simulink model "lab5_control"  (R2026a)
settings: Solver=ode4  StopTime=T_FIN  FixedStep=1e-4
PreLoadFcn:
  | run(fullfile(fileparts(get_param(bdroot,'FileName')),'parametros.m'));
InitFcn:
  | run(fullfile(fileparts(get_param(bdroot,'FileName')),'parametros.m'));
values from neighbouring files (symbols this model uses):
  a0 = 622.9    [parametros.m]
  a1 = 46.87    [parametros.m]
  b0 = 168.4    [parametros.m]
  Kd = (Pd_s(2) - a1)/b0    [parametros.m]
  Ki = Pd_s(4)/b0    [parametros.m]
  Kp = (Pd_s(3) - a0)/b0    [parametros.m]
  q0_cd = Kd/T + Kp + Ki*T    [parametros.m]
  q0_dd = sol(1)    [parametros.m]
  q1_cd = -2*Kd/T - Kp    [parametros.m]
  q1_dd = sol(2)    [parametros.m]
  q2_cd = Kd/T    [parametros.m]
  q2_dd = sol(3)    [parametros.m]
  R1 = 5    [parametros.m]
  R2 = -5    [parametros.m]
  s0_cd = 0    [parametros.m]
  s0_dd = sol(4)    [parametros.m]
  T = 0.01    [parametros.m]
  T_R1 = 0.1    [parametros.m]
  T_R2 = 1.6    [parametros.m]
  U_MAX = 100 - U0_POS    (= 57.9)    [parametros.m]
  U_MIN = -(100 - U0_NEG)    (= -44.7)    [parametros.m]
settings Model: Creator=PERSONAL  LastModifiedBy=PERSONAL

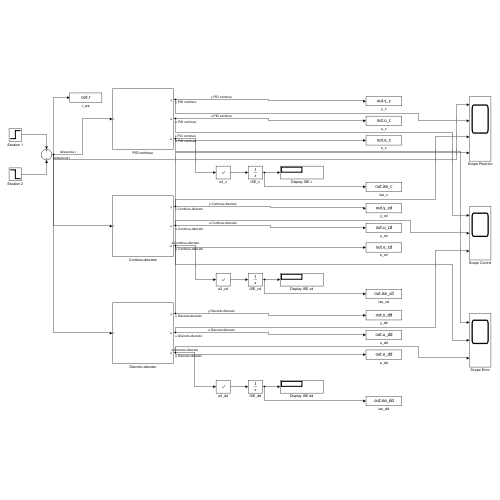
[thumbnail: Simulink's stored preview of the top-level diagram]
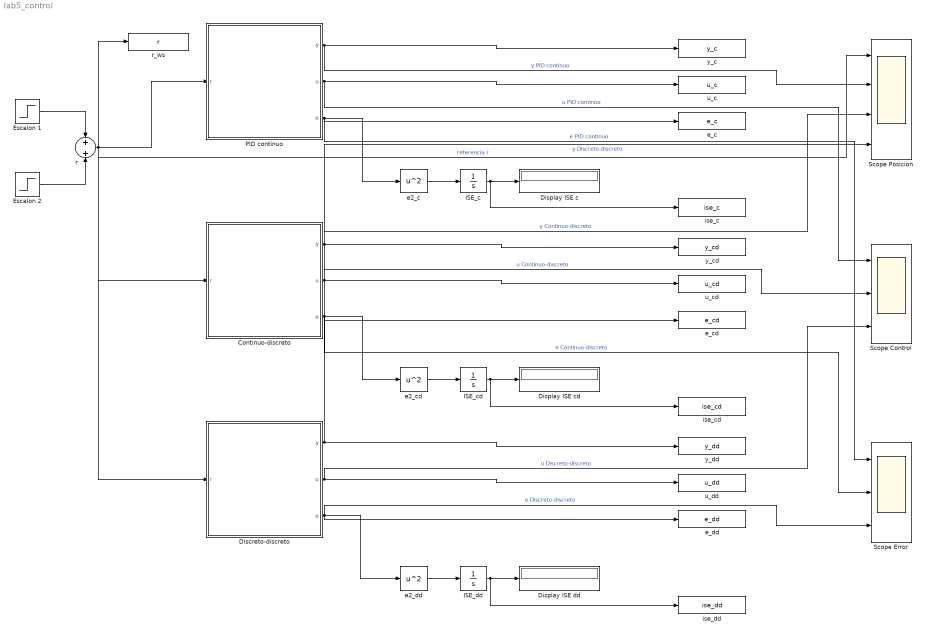
== system lab5_control ==
  Continuo-discreto : Subsystem
  Discreto-discreto : Subsystem
  Display ISE c : Display
  Display ISE cd : Display
  Display ISE dd : Display
  Escalon 1 : Step  Time=T_R1  FinalValue=R1  SampleTime=0
  Escalon 2 : Step  Time=T_R2  FinalValue=R2-R1  SampleTime=0
  ISE_c : Integrator
  ISE_cd : Integrator
  ISE_dd : Integrator
  PID continuo : Subsystem
  Scope Control : Scope  NumInputPorts=3
  Scope Error : Scope  NumInputPorts=3
  Scope Posicion : Scope  NumInputPorts=4
  e2_c : Math  Operator=square
  e2_cd : Math  Operator=square
  e2_dd : Math  Operator=square
  e_c : ToWorkspace  VariableName=e_c  SaveFormat=Timeseries  SampleTime=1e-3
  e_cd : ToWorkspace  VariableName=e_cd  SaveFormat=Timeseries  SampleTime=1e-3
  e_dd : ToWorkspace  VariableName=e_dd  SaveFormat=Timeseries  SampleTime=1e-3
  ise_c : ToWorkspace  VariableName=ise_c  SaveFormat=Timeseries  SampleTime=1e-3
  ise_cd : ToWorkspace  VariableName=ise_cd  SaveFormat=Timeseries  SampleTime=1e-3
  ise_dd : ToWorkspace  VariableName=ise_dd  SaveFormat=Timeseries  SampleTime=1e-3
  r : Sum
  r_ws : ToWorkspace  VariableName=r  SaveFormat=Timeseries  SampleTime=1e-3
  u_c : ToWorkspace  VariableName=u_c  SaveFormat=Timeseries  SampleTime=1e-3
  u_cd : ToWorkspace  VariableName=u_cd  SaveFormat=Timeseries  SampleTime=1e-3
  u_dd : ToWorkspace  VariableName=u_dd  SaveFormat=Timeseries  SampleTime=1e-3
  y_c : ToWorkspace  VariableName=y_c  SaveFormat=Timeseries  SampleTime=1e-3
  y_cd : ToWorkspace  VariableName=y_cd  SaveFormat=Timeseries  SampleTime=1e-3
  y_dd : ToWorkspace  VariableName=y_dd  SaveFormat=Timeseries  SampleTime=1e-3
  wires:
  Discreto-discreto/2(u) -> u_dd/1, Scope Control/3  "u Discreto-discreto"
  Discreto-discreto/1(y) -> y_dd/1, Scope Posicion/4  "y Discreto-discreto"
  ISE_dd/1 -> Display ISE dd/1, ise_dd/1
  e2_dd/1 -> ISE_dd/1
  Discreto-discreto/3(e) -> e2_dd/1, e_dd/1, Scope Error/3  "e Discreto-discreto"
  Continuo-discreto/2(u) -> u_cd/1, Scope Control/2  "u Continuo-discreto"
  Continuo-discreto/1(y) -> y_cd/1, Scope Posicion/3  "y Continuo-discreto"
  ISE_cd/1 -> Display ISE cd/1, ise_cd/1
  e2_cd/1 -> ISE_cd/1
  Continuo-discreto/3(e) -> e2_cd/1, e_cd/1, Scope Error/2  "e Continuo-discreto"
  PID continuo/2(u) -> u_c/1, Scope Control/1  "u PID continuo"
  PID continuo/1(y) -> y_c/1, Scope Posicion/2  "y PID continuo"
  ISE_c/1 -> Display ISE c/1, ise_c/1
  e2_c/1 -> ISE_c/1
  PID continuo/3(e) -> e2_c/1, e_c/1, Scope Error/1  "e PID continuo"
  r/1 -> PID continuo/1(r), Continuo-discreto/1(r), Discreto-discreto/1(r), r_ws/1, Scope Posicion/1  "referencia r"
  Escalon 2/1 -> r/2
  Escalon 1/1 -> r/1

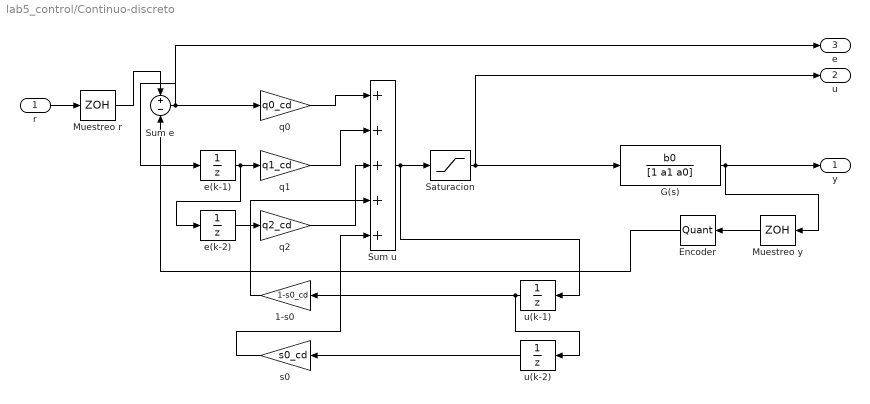
== system lab5_control/Continuo-discreto ==
  r : Inport
  1-s0 : Gain  Gain=1-s0_cd
  Encoder : Quantizer  QuantizationInterval=Q_ENC
  G(s) : TransferFcn  Numerator=b0  Denominator=[1 a1 a0]
  Muestreo r : ZeroOrderHold  SampleTime=T
  Muestreo y : ZeroOrderHold  SampleTime=T
  Saturacion : Saturate  UpperLimit=U_MAX  LowerLimit=U_MIN
  Sum e : Sum  Inputs=+-
  Sum u : Sum  Inputs=+++++
  e(k-1) : UnitDelay  SampleTime=T
  e(k-2) : UnitDelay  SampleTime=T
  q0 : Gain  Gain=q0_cd
  q1 : Gain  Gain=q1_cd
  q2 : Gain  Gain=q2_cd
  s0 : Gain  Gain=s0_cd
  u(k-1) : UnitDelay  SampleTime=T
  u(k-2) : UnitDelay  SampleTime=T
  y : Outport
  u : Outport  Port=2
  e : Outport  Port=3
  wires:
  r/1 -> Muestreo r/1
  Muestreo r/1 -> Sum e/1
  Sum e/1 -> q0/1, e(k-1)/1, e/1
  e(k-1)/1 -> q1/1, e(k-2)/1
  e(k-2)/1 -> q2/1
  q0/1 -> Sum u/1
  q1/1 -> Sum u/2
  q2/1 -> Sum u/3
  1-s0/1 -> Sum u/4
  s0/1 -> Sum u/5
  Sum u/1 -> Saturacion/1, u(k-1)/1
  Saturacion/1 -> G(s)/1, u/1
  u(k-1)/1 -> 1-s0/1, u(k-2)/1
  u(k-2)/1 -> s0/1
  G(s)/1 -> y/1, Muestreo y/1
  Muestreo y/1 -> Encoder/1
  Encoder/1 -> Sum e/2

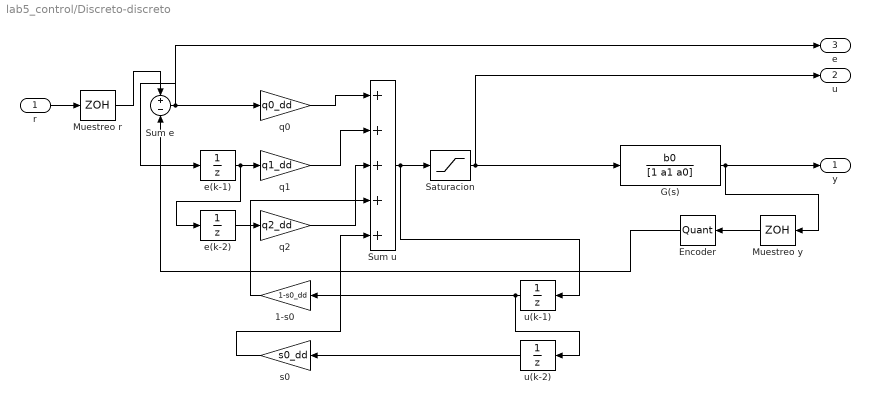
== system lab5_control/Discreto-discreto ==
  r : Inport
  1-s0 : Gain  Gain=1-s0_dd
  Encoder : Quantizer  QuantizationInterval=Q_ENC
  G(s) : TransferFcn  Numerator=b0  Denominator=[1 a1 a0]
  Muestreo r : ZeroOrderHold  SampleTime=T
  Muestreo y : ZeroOrderHold  SampleTime=T
  Saturacion : Saturate  UpperLimit=U_MAX  LowerLimit=U_MIN
  Sum e : Sum  Inputs=+-
  Sum u : Sum  Inputs=+++++
  e(k-1) : UnitDelay  SampleTime=T
  e(k-2) : UnitDelay  SampleTime=T
  q0 : Gain  Gain=q0_dd
  q1 : Gain  Gain=q1_dd
  q2 : Gain  Gain=q2_dd
  s0 : Gain  Gain=s0_dd
  u(k-1) : UnitDelay  SampleTime=T
  u(k-2) : UnitDelay  SampleTime=T
  y : Outport
  u : Outport  Port=2
  e : Outport  Port=3
  wires:
  r/1 -> Muestreo r/1
  Muestreo r/1 -> Sum e/1
  Sum e/1 -> q0/1, e(k-1)/1, e/1
  e(k-1)/1 -> q1/1, e(k-2)/1
  e(k-2)/1 -> q2/1
  q0/1 -> Sum u/1
  q1/1 -> Sum u/2
  q2/1 -> Sum u/3
  1-s0/1 -> Sum u/4
  s0/1 -> Sum u/5
  Sum u/1 -> Saturacion/1, u(k-1)/1
  Saturacion/1 -> G(s)/1, u/1
  u(k-1)/1 -> 1-s0/1, u(k-2)/1
  u(k-2)/1 -> s0/1
  G(s)/1 -> y/1, Muestreo y/1
  Muestreo y/1 -> Encoder/1
  Encoder/1 -> Sum e/2

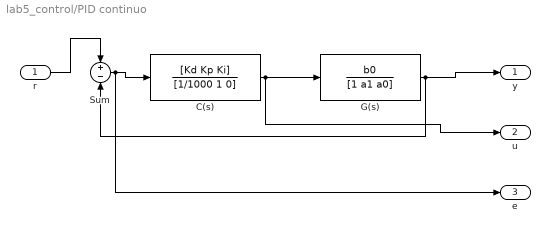
== system lab5_control/PID continuo ==
  r : Inport
  C(s) : TransferFcn  Numerator=[Kd Kp Ki]  Denominator=[1/1000 1 0]
  G(s) : TransferFcn  Numerator=b0  Denominator=[1 a1 a0]
  Sum : Sum  Inputs=+-
  y : Outport
  u : Outport  Port=2
  e : Outport  Port=3
  wires:
  r/1 -> Sum/1
  Sum/1 -> C(s)/1, e/1
  C(s)/1 -> G(s)/1, u/1
  G(s)/1 -> y/1, Sum/2
